simulink model "engine"  (R2021b)
settings: Solver=VariableStepAuto  StartTime=0.0  StopTime=20  RelTol=1e-3
settings Model: Creator=Jihoon Lee  LastModifiedBy=Jihoon Lee

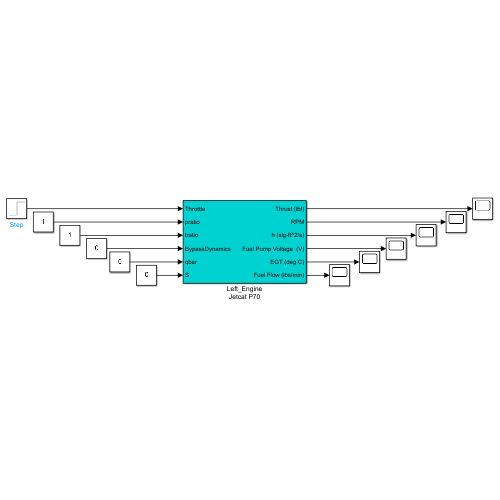
[thumbnail: Simulink's stored preview of the top-level diagram]
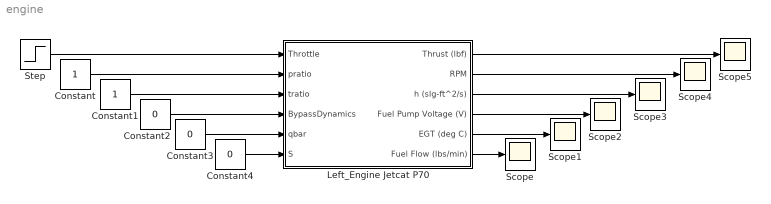
== system engine ==
  Constant : Constant
  Constant1 : Constant
  Constant2 : Constant  Value=0
  Constant3 : Constant  Value=0
  Constant4 : Constant  Value=0
  Left_Engine Jetcat P70 : Subsystem
      mask init:
      | % Curve fit parameters for Jetcat P70 Model
      | % Coeff_thrust   = [0.000028864242464  -0.001914835880159 0.105916926095459  -1.251646340183624 ];
      | Coeff_thrust   = [0.000014847593013,  0, 0, 0.412662356277121];
      | Coeff_throttle = [0.000033035538475  -0.008354385314499 1.191126728328792 31.518959847101669];
      | Coeff_fuelflow = [0.000046800927870  -0.000779344124807 0.122178501497750];
      | Coeff_tau      = [ -2.2400e-02   2.9948e+00];
      | Coeff_EGT      = [ 2E-5, -0.0036,0.2342,-8.0496,664.99]; %EGT model, deg C
      | Coeff_dynamics = [ -.074 7.1];
      | fuelpump_table = [0 0.576	0.625	0.6985	0.7845	0.8575	0.919	0.9805	1.0415	1.1025...
      |                     1.1515	1.262	1.287	1.373	1.52	1.618	1.74	1.887	1.973...
      |                     2.12	2.255	2.4385	2.647	2.7575	2.9905	3.162]; %volts, table of fuel pump voltages
      | fuelflow_table = [0,0.0794,0.0876,0.102,0.1149,0.1275,0.1379,0.1487,0.1586,0.1671,...
      |                     0.1775,0.1858,0.194,0.2038,0.2206,0.2405,0.2566,0.2746,0.2921,0.3102,...
      |                     0.3266,0.3445,0.3533,0.3611,0.3866,0.4083;]*2; %lbs/min,   FULL fuel flow rates corresponding to pump voltages (fuelpump_table)  
      | % Equvalent Shaft parameters for engine
      | shaft_dia = 0.75/12.0;       % diameter of rotating turbine in feet 
      | shaft_len = 6.25/12.0;       % length of rotating turbine in feet   
      | density   = 15.2;            % mass density of steel in slugs/ft^3 
      | 
      | 
      | A = [-1.336,-0.7314;1,0;];
      | B = [1;0];
      | C = [-0.1474   0.7314];
      | D = 0;
  Scope{,1..5} (6 alike) : Scope
  Step : Step  After=100  SampleTime=0
  wires:
  Step/1 -> Left_Engine Jetcat P70/1(Throttle)
  Constant/1 -> Left_Engine Jetcat P70/2(pratio)
  Constant1/1 -> Left_Engine Jetcat P70/3(tratio)
  Constant2/1 -> Left_Engine Jetcat P70/4(BypassDynamics)
  Constant3/1 -> Left_Engine Jetcat P70/5(qbar)
  Constant4/1 -> Left_Engine Jetcat P70/6(S)
  Left_Engine Jetcat P70/6(Fuel Flow (lbs/min)) -> Scope/1
  Left_Engine Jetcat P70/5(EGT (deg C)) -> Scope1/1
  Left_Engine Jetcat P70/4(Fuel Pump Voltage (V)) -> Scope2/1
  Left_Engine Jetcat P70/3(h (slg-ft^2/s)) -> Scope3/1
  Left_Engine Jetcat P70/2(RPM) -> Scope4/1
  Left_Engine Jetcat P70/1(Thrust (lbf)) -> Scope5/1

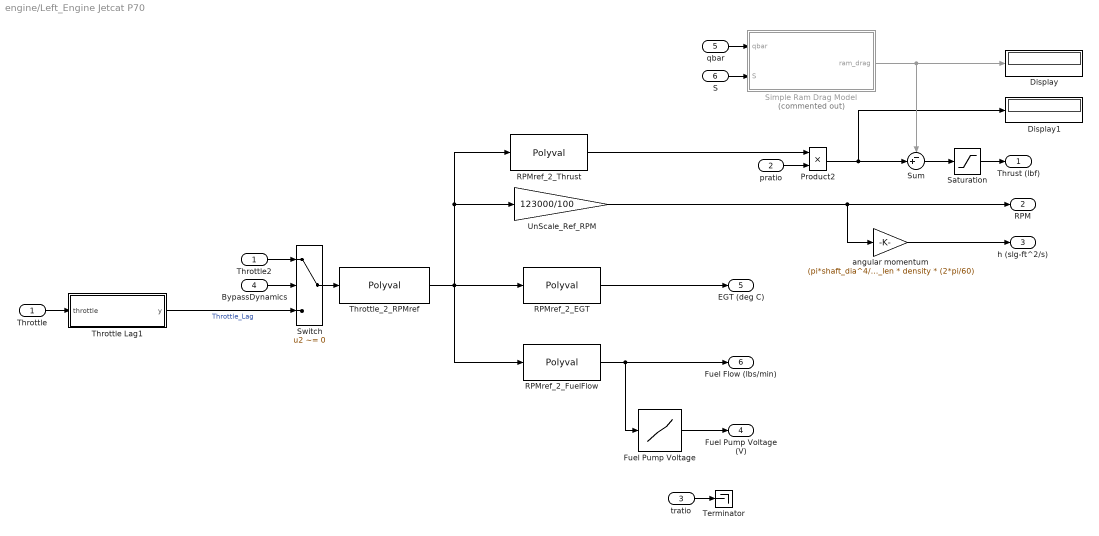
== system engine/Left_Engine Jetcat P70 ==
  Throttle : Inport
  pratio : Inport  Port=2
  tratio : Inport  Port=3
  BypassDynamics : Inport  Port=4
  qbar : Inport  Port=5
  S : Inport  Port=6
  Display : Display
  Display1 : Display
  Fuel Pump Voltage : Lookup  InputValues=fuelflow_table  Table=fuelpump_table  LookUpMeth=Interpolation-Use End Values
  Product2 : Product  RndMeth=Zero
  RPMref_2_EGT : Polyval  Coefs=Coeff_EGT
  RPMref_2_FuelFlow : Polyval  Coefs=Coeff_fuelflow
  RPMref_2_Thrust : Polyval  Coefs=Coeff_thrust
  Saturation : Saturate  UpperLimit=inf  LowerLimit=0
  Simple Ram Drag Model : MATLAB Function  Commented=on  TreatAsAtomicUnit=on
  Sum : Sum  Inputs=-+|
  Switch : Switch  Criteria=u2 ~= 0
  Terminator : Terminator
  Throttle Lag1 : Subsystem
  Throttle2 : InportShadow
  Throttle_2_RPMref : Polyval  Coefs=Coeff_throttle
  UnScale_Ref_RPM : Gain  Gain=123000/100
  angular momentum : Gain  Gain=(pi*shaft_dia^4/32) * shaft_len * density * (2*pi/60)
  Thrust (lbf) : Outport
  RPM : Outport  Port=2
  h (slg-ft^2/s) : Outport  Port=3
  Fuel Pump Voltage (V) : Outport  Port=4
  EGT (deg C) : Outport  Port=5
  Fuel Flow (lbs/min) : Outport  Port=6
  wires:
  Saturation/1 -> Thrust (lbf)/1
  Sum/1 -> Saturation/1
  Product2/1 -> Display1/1, Sum/2
  Simple Ram Drag Model/1(ram_drag) -> Sum/1, Display/1
  S/1 -> Simple Ram Drag Model/2(S)
  qbar/1 -> Simple Ram Drag Model/1(qbar)
  Throttle2/1 -> Switch/1
  BypassDynamics/1 -> Switch/2
  Throttle Lag1/1(y) -> Switch/3  "Throttle_Lag"
  Switch/1 -> Throttle_2_RPMref/1
  Throttle/1 -> Throttle Lag1/1(throttle)
  Throttle_2_RPMref/1 -> RPMref_2_Thrust/1, UnScale_Ref_RPM/1, RPMref_2_EGT/1, RPMref_2_FuelFlow/1
  angular momentum/1 -> h (slg-ft^2/s)/1
  UnScale_Ref_RPM/1 -> angular momentum/1, RPM/1
  tratio/1 -> Terminator/1
  RPMref_2_Thrust/1 -> Product2/1
  RPMref_2_FuelFlow/1 -> Fuel Flow (lbs/min)/1, Fuel Pump Voltage/1
  pratio/1 -> Product2/2
  Fuel Pump Voltage/1 -> Fuel Pump Voltage (V)/1
  RPMref_2_EGT/1 -> EGT (deg C)/1

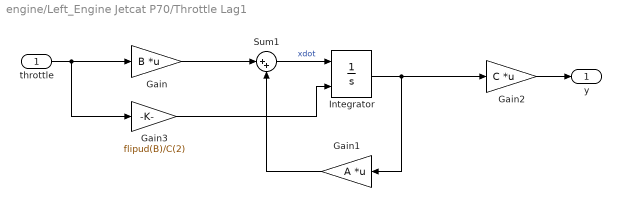
== system engine/Left_Engine Jetcat P70/Throttle Lag1 ==
  throttle : Inport
  Gain : Gain  Gain=B  Multiplication=Matrix(K*u)
  Gain1 : Gain  Gain=A  Multiplication=Matrix(K*u)
  Gain2 : Gain  Gain=C  Multiplication=Matrix(K*u)
  Gain3 : Gain  Gain=flipud(B)/C(2)
  Integrator : Integrator  InitialConditionSource=external
  Sum1 : Sum  Inputs=|++
  y : Outport
  wires:
  Sum1/1 -> Integrator/1  "xdot"
  Gain1/1 -> Sum1/2
  Integrator/1 -> Gain1/1, Gain2/1
  Gain/1 -> Sum1/1
  Gain2/1 -> y/1
  throttle/1 -> Gain/1, Gain3/1
  Gain3/1 -> Integrator/2

== matlab function engine/Left_Engine Jetcat P70/Simple Ram Drag Model ==
  data: ram_drag output; qbar input; S input; ram_drag_coef parameter
function ram_drag =   ram_drag(qbar,S,ram_drag_coef)
% This block supports the Embedded MATLAB subset.
% See the help menu for details. 

ram_drag = ram_drag_coef.*qbar.*S;
return
